simulink subsystem "theta_el_Calc"  (R2025b)
settings: Solver=VariableStepAuto  StartTime=0.0  StopTime=10.0  RelTol=1e-3
undefined symbols (not defined in the file): FOC, Plant
settings Model: Creator=kara  LastModifiedBy=kara
settings RTWCC: GPUComputeCapability=3.5

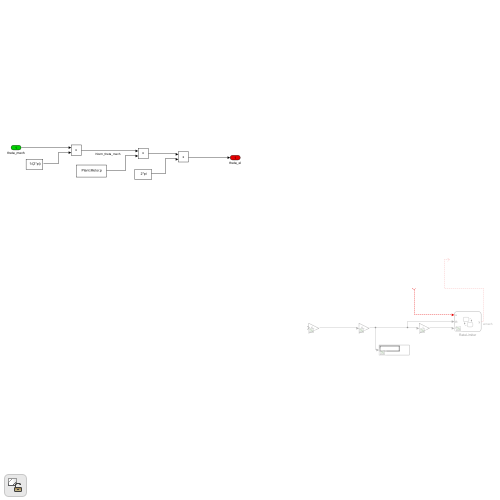
[thumbnail: Simulink's stored preview of the top-level diagram]
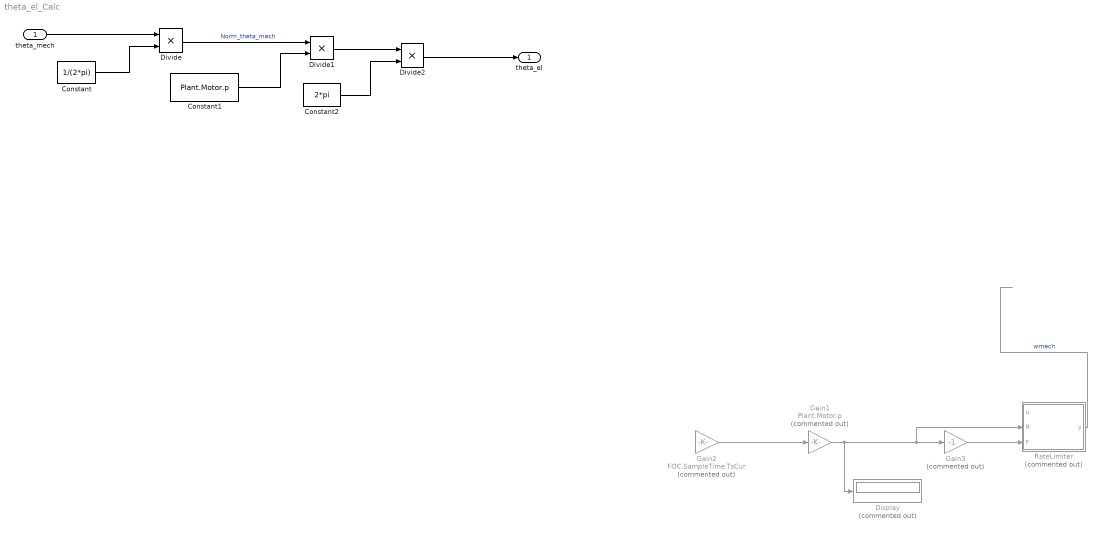
== system theta_el_Calc ==
  theta_mech : Inport
  Constant : Constant  Value=1/(2*pi)  OutDataTypeStr=PWMGenSacling
  Constant1 : Constant  Value=Plant.Motor.p  OutDataTypeStr=uint8
  Constant2 : Constant  Value=2*pi  OutDataTypeStr=UHighScaling
  Display : Display  Commented=on
  Divide : Product  Inputs=**  OutDataTypeStr=fixdt(0,32,32)
  Divide1 : Product  Inputs=**  OutDataTypeStr=fixdt(0,32,32)
  Divide2 : Product  Inputs=**  OutDataTypeStr=HighScaling
  Gain1 : Gain  Commented=on  Gain=Plant.Motor.p  OutDataTypeStr=HighScaling
  Gain2 : Gain  Commented=on  Gain=FOC.SampleTime.TsCur  OutDataTypeStr=FineScaling
  Gain3 : Gain  Commented=on  Gain=-1  OutDataTypeStr=HighScaling
  RateLimiter : Stateflow chart  Commented=on  TreatAsAtomicUnit=on
  theta_el : Outport
  wires:
  Constant2/1 -> Divide2/2
  Divide1/1 -> Divide2/1
  Divide2/1 -> theta_el/1
  ? -> RateLimiter/1(u)
  RateLimiter/1(y) -> ?  "wmech"
  Gain3/1 -> RateLimiter/3(F)
  Gain1/1 -> Display/1, RateLimiter/2(R), Gain3/1
  Gain2/1 -> Gain1/1
  theta_mech/1 -> Divide/1
  Divide/1 -> Divide1/1  "Norm_theta_mech"
  Constant1/1 -> Divide1/2
  Constant/1 -> Divide/2

== stateflow chart theta_el_Calc/RateLimiter ==
  settings: updateMethod=DISCRETE  sampleTime=FOC.SampleTime.TsCur
  state IDLE
  state Rising
    entry:  y =  fi(y_prev +dT * R, 1, 32, 27);
    exit: y_prev = y;
  state Falling
    entry:  y = fi(y_prev+dT * F, 1, 32, 27);
    exit: y_prev = y;
  state Directpassage
    entry:  y = u;
    exit: y_prev = y;
  (default) -> IDLE
  IDLE -> (junction 22)
  (junction 22) -> Rising [order 1] : [(u-y_prev)/dT>=R]
  (junction 22) -> Falling [order 2] : [(u-y_prev)/dT<=F]
  Rising -> (junction 22)
  Falling -> (junction 22)
  Directpassage -> (junction 22)
  (junction 22) -> Directpassage [order 3] : [(u-y_prev)/dT<R && (u-y_prev)/dT>F]
  data: u input HighScaling; R input HighScaling; F input HighScaling; dT constant HighScaling size=1 =FOC.SampleTime.TsCur; y output HighScaling; y_prev local HighScaling =0
